simulink model "export_to_stm"  (R2026a)
settings: Solver=FixedStepAuto  EnableMultiTasking=on
values from neighbouring files (symbols this model uses):
  Ts = 1.0E-6    [vars.sldd]
undefined symbols (not defined in the file or in its folder): bits
libraries: stm32f4xxblockslib x2, slpidlib x1, stm32blockslib x1
settings Model: DataDictionary=vars.sldd  STM32="{\"AnalogInput\":{\"ID\":\"60\"},\"I2CControllerRead\":{\"ID\":\"62\"},\"PWMOutput\":{\"ID\":\"63\"}}"  Creator=caden  LastModifiedBy=caden
settings HardwareCC: ProdLargestAtomicInteger=Long  ProdLargestAtomicFloat=Double  ProdHWDeviceType=ARM Compatible->ARM Cortex-M
settings RTWCC: SystemTargetFile=ert.tlc  HardwareBoard=STM32G4xx Based  TLCOptions=-aInlineSetEventsForThisBaseRateFcn=TLC_FALSE -aSuppressMultiTaskScheduler=TLC_FALSE -aRateBasedStepFcn=1  Toolchain=GNU Tools for STM32  BuildConfiguration=Faster Runs  Description=Embedded Coder
settings ERTTargetCC: ExtModeTransport=3.0  ExtModeStaticAllocSize=2048.0  CodeReplacementLibrary=ARM Cortex-M

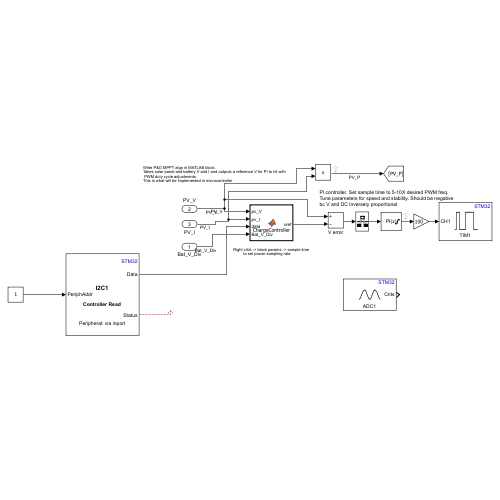
[thumbnail: Simulink's stored preview of the top-level diagram]
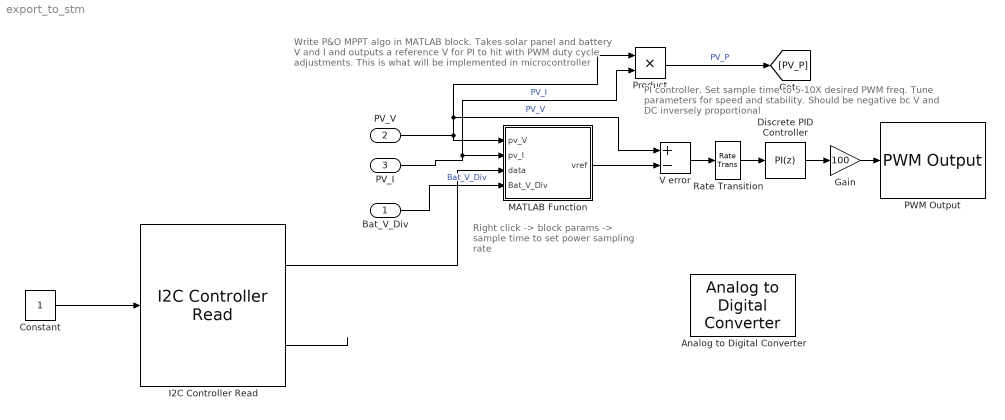
== system export_to_stm ==
  note: PI controller. Set sample time to 5-10X desired PWM freq.
      | Tune parameters for speed and stability. Should be negative
      | bc V and DC inversely proportional
  note: Right click -> block params -> sample time
      | to set power sampling rate
  note: Write P&O MPPT algo in MATLAB block.
      | Takes solar panel and battery V and I and outputs a reference V for PI to hit with
      | PWM duty cycle adjustments.
      | This is what will be implemented in microcontroller
  Bat_V_Div : Inport
  PV_V : Inport  Port=2  SampleTime=Ts
  PV_I : Inport  Port=3  SampleTime=Ts
  Analog to Digital Converter : stm32f4xxblockslib/Analog to Digital Converter  ADCModule=ADC1  ConversionGroup=Regular  TriggerMode=Trigger and read  NumberOfConversions=1  EnableBufferConv=off  BufferLength=1  OutputStatus=off  SampleTime=-1  EnableSimPort=off  hoistedMaskSrc=ECSoC/ECSimCodegen/Analog to Digital Converter
  Constant : Constant
  Discrete PID Controller : slpidlib/PID Controller  Controller=PI  Form=Parallel  TimeDomain=Discrete-time  UseExternalTs=off  SampleTime=1e-4  IntegratorMethod=Backward Euler  FilterMethod=Forward Euler  ControllerParametersSource=internal  P=0.005  I=0.0002  UseKiTs=on  D=0  UseExternalDerivativeSource=off  N=100  UseFilter=on  TunerSelectOption=Transfer Function Based (PID Tuner App)  InitialConditionSource=internal  InitialConditionForIntegrator=0.5  InitialConditionForFilter=0  DifferentiatorICPrevScaledInput=0  ExternalReset=none  TrackingMode=off  Kt=1  LimitOutput=on  SatLimitsSource=internal  UpperSaturationLimit=0.95  LowerSaturationLimit=0.05  LinearizeAsGain=off  AntiWindupMode=none  Kb=1  LimitIntegrator=on  UpperIntegratorSaturationLimit=0.95  LowerIntegratorSaturationLimit=0.05  POutMin=[]  POutMax=[]  IOutMin=[]  IOutMax=[]  DOutMin=[]  DOutMax=[]  NOutMin=[]  NOutMax=[]  SumOutMin=[]  SumOutMax=[]  SaturationOutMin=[]  SaturationOutMax=[]  PParamMin=[]  PParamMax=[]  IParamMin=[]  IParamMax=[]  DParamMin=[]  DParamMax=[]  NParamMin=[]  NParamMax=[]  KbParamMin=[]  KbParamMax=[]  KtParamMin=[]  KtParamMax=[]  KbOutMin=[]  KbOutMax=[]  KtOutMin=[]  KtOutMax=[]  IntegratorOutMin=[]  IntegratorOutMax=[]  FilterOutMin=[]  FilterOutMax=[]  SumI1OutMin=[]  SumI1OutMax=[]  SumI2OutMin=[]  SumI2OutMax=[]  SumI3OutMin=[]  SumI3OutMax=[]  SumI4OutMin=[]  SumI4OutMax=[]  SumDOutMin=[]  SumDOutMax=[]  DifferentiatorOutMin=[]  DifferentiatorOutMax=[]  FilterDiffOutCoefMin=[]  FilterDiffOutCoefMax=[]  ReciprocalOutMin=[]  ReciprocalOutMax=[]  SumDenOutMin=[]  SumDenOutMax=[]  SumNumOutMin=[]  SumNumOutMax=[]  DivideOutMin=[]  DivideOutMax=[]  UdiffTsProdOutMin=[]  UdiffTsProdOutMax=[]  NTsProdOutMin=[]  NTsProdOutMax=[]  UintegralTsProdOutMin=[]  UintegralTsProdOutMax=[]  UngainTsProdOutMin=[]  UngainTsProdOutMax=[]  ClampingZeroOutDataTypeStr=Inherit: Inherit via back propagation  ClampingZeroOutMin=[]  ClampingZeroOutMax=[]  FilterDenConstantOutDataTypeStr=Inherit: Inherit via back propagation  FilterDenConstantOutMin=[]  FilterDenConstantOutMax=[]  PCopyOutDataTypeStr=Inherit: Inherit via back propagation  PCopyOutMin=[]  PCopyOutMax=[]  NCopyOutDataTypeStr=Inherit: Inherit via back propagation  NCopyOutMin=[]  NCopyOutMax=[]  IntegratorContinuousStateAttributes=''  IntegratorStateMustResolveToSignalObject=off  IntegratorRTWStateStorageClass=Auto  FilterContinuousStateAttributes=''  FilterStateMustResolveToSignalObject=off  FilterRTWStateStorageClass=Auto  ParallelPVariant=InternalParameters  IdealPVariant=Disabled  IVariant=InternalParameters  DVariant=Disabled  IntegratorVariant=Discrete  SatVariant=Enabled  AWVariant=Passthrough  PCopyVariant=Disabled  TRVariant=Disabled  FdbkBlocksVariant=Forward  IdealPFdbkVariant=Disabled  SatFdbkVariant=Disabled  DerivativeFilterVariant=Disabled  NVariant=Disabled  NCopyVariant=Disabled_SignalSpec  FilterICVariant=Disabled  IntegratorICVariant=InternalICs  ExternalResetVariant=Disabled  TRSumVariant=Passthrough  SumFdbkVariant=Disabled  SumVariant=Sum_PI  TsampFilterVariant=InternalTs  TsampNgainVariant=Passthrough  TsampIntegralVariant=Disabled_SignalSpec  ExternalSaturationOutDataTypeStr=Inherit: Same as second input  DerivativeSourceVariant=Disabled  PreIntVariant=InternalPreInt
      settings: LibrarySourceBlock=simulink/Discrete/Discrete PID Controller
  Gain : Gain  Gain=100
  I2C Controller Read : stm32blockslib/I2C Controller Read  I2CModule=I2C1  Mode=Controller  AddressingMode=7-bits  PeripheralByteOrder=BigEndian  OwnPeripheralAddress=uint8(170)  PeripheralAddressVia=Inport  PeripheralAddress=10  RegisterAddressMode=on  RegisterAddressVia=Dialog  RegisterAddress=1  RepeatedStart=off  NoAck=off  OutputStatus=on  BlockMode=Receive  DataType=uint8  DataLength=1  Timeout=0.001  SampleTime=-1
      settings: LibrarySourceBlock=stm32g4xxblockslib/I2C Controller Read
  MATLAB Function : MATLAB Function  TreatAsAtomicUnit=on  SystemSampleTime=0.01
  PWM Output : stm32f4xxblockslib/PWM Output  ProcessorFamily=STM32G4  TimerModule=TIM1  DutycycleUnits=Percentage  EnableChannel1=on  EnableCaptureCompare1Input=off  EnableCaptureCompare1ComplementaryInput=off  EnableOutputCompare1ModeInput=off  EnableChannel2=off  EnableCaptureCompare2Input=off  EnableCaptureCompare2ComplementaryInput=off  EnableOutputCompare2ModeInput=off  EnableChannel3=off  EnableCaptureCompare3Input=off  EnableCaptureCompare3ComplementaryInput=off  EnableOutputCompare3ModeInput=off  EnableChannel4=off  EnableCaptureCompare4Input=off  EnableCaptureCompare4ComplementaryInput=off  EnableOutputCompare4ModeInput=off  EnableChannel5=off  EnableCaptureCompare5Input=off  EnableOutputCompare5ModeInput=off  EnableChannel6=off  EnableCaptureCompare6Input=off  EnableOutputCompare6ModeInput=off  EnableCounterInput=off  EnableMainOutputInput=off  EnableFrequencyInput=off  SetRCAfterCE=off  OutputDirection=off  OutputMainOutputEnableStatus=off  SampleTime=0.1  EnableSimPort=off  EnableUpdateEvent=off  EnableCaptureCompare1Event=off  EnableCaptureCompare2Event=off  EnableCaptureCompare3Event=off  EnableCaptureCompare4Event=off  EnableTriggerEvent=off  EnableBreakEvent=off  EnableBreakEvent2=off  hoistedMaskSrc=ECSoC/ECSimCodegen/PWM Output
      settings: LibrarySourceBlock=stm32g4xxblockslib/PWM Output
  Product : Product
  Rate Transition : RateTransition
  V error : Sum  Inputs=+-
  wires:
  Rate Transition/1 -> Discrete PID Controller/1
  V error/1 -> Rate Transition/1
  Product/1 -> [PV_P]  "PV_P"
  MATLAB Function/1(vref) -> V error/2
  PV_V/1 -> MATLAB Function/1(pv_V), V error/1, Product/1  "PV_V"
  Bat_V_Div/1 -> MATLAB Function/4(Bat_V_Div)  "Bat_V_Div"
  PV_I/1 -> MATLAB Function/2(pv_I), Product/2  "PV_I"
  Discrete PID Controller/1 -> Gain/1
  Gain/1 -> PWM Output/1
  I2C Controller Read/2 -> ?
  I2C Controller Read/1 -> MATLAB Function/3(data)
  Constant/1 -> I2C Controller Read/1

== matlab function export_to_stm/MATLAB Function ==
  data: pv_V input; vref output; pv_I input; data input; Bat_V_Div input
% 3 charge states: 
% 1. Bulk (mppt): battery low or mid. Route max power
% 2. Absorption: battery nearly full, stop MPPT and hold V at high level
% 3. Float: Battery 100% charged. Sit at slightly lower V to maintain
% charge w/o overcharging
function vref = ChargeController(pv_V,pv_I,data, Bat_V_Div)
    persistent charge_state P_old V_mpp_tracked;
    V_DIV_RATIO = 5; %Set to (Big R + Small R)/Small R of bat V divider
    bat_V = Bat_V_Div * V_DIV_RATIO; %This should recover the bat's actual V
    V_STEP = 0.02; % Tune me!
    V_MAX = 22;%21.8; %Voc
    V_MIN = 12.0;
    V_ABSORPTION = 14.4; %battery voltage when full
    V_FLOAT = 13.5; %Maintenance V, prevent overcharge
    V_INITIAL_GUESS = 18; %Best to guess operating voltage initially


   
   
   
   % INITIAL (BOOT)
   if isempty(charge_state)
        charge_state = 1; %bulk
        V_mpp_tracked = V_INITIAL_GUESS; %Guess the initial voltage to track (rated V)
        P_old = 0;
   end
   pv_P = pv_V * pv_I; %Current panel power

   %CHARGING STATE MACHINE
   if charge_state == 1 % 1. BULK
        if bat_V >= V_ABSORPTION %Close to full?
            charge_state = 2; %enter absorption state
            vref = V_mpp_tracked;
        else %do P&O
            vref = Piano(pv_V, pv_P, V_mpp_tracked, P_old, V_STEP, V_MAX, V_MIN);
            V_mpp_tracked = vref;
            P_old = pv_P;
        end

   elseif charge_state == 2 % 2. ABSORPTION (80-85% full)
        if bat_V >= (V_ABSORPTION + 0.1) % Battery V too high
            vref = V_mpp_tracked + V_STEP; % Increase pv voltage
        elseif bat_V < V_ABSORPTION       % Battery V too low
            vref = V_mpp_tracked - V_STEP;  % Decrease pv voltage
        else     % Battery V good
            vref = V_mpp_tracked;
        end

   else % 3. FLOAT (~100% full)
       if bat_V >= (V_FLOAT + 0.1) % Battery V too high
           vref = V_mpp_tracked + V_STEP; % Increase pv voltage
       elseif bat_V < V_FLOAT       % Battery V too low
           vref = V_mpp_tracked - V_STEP;  % Decrease pv voltage
       else     % Battery V good
           vref = V_mpp_tracked;
       end
        % I don't know how to implement transition to/from float yet.
        % Can use timer (~1hr) or track battery current to decide when full
   end
   
end

%---MPPT----
% Perturb & Observe (P&O)
function vref_out = Piano(pv_V, pv_P, V_old, P_old, v_step, v_max, v_min)
    
    dP = pv_P-P_old;
    dV = pv_V-V_old;
    if dP > 0
        if dV > 0
            vref_out = V_old + v_step;
        else
            vref_out = V_old - v_step;
        end
    else
        if dV > 0
            vref_out = V_old - v_step;
        else
            vref_out = V_old + v_step;
        end
    end

    % Boundaries
    vref_out = max(v_min, min(v_max,vref_out));
end
